simulink model "AlphaBotOdometrie"  (R2026b)
settings: Solver=FixedStepDiscrete  StopTime=inf  FixedStep=PAR_Sys_AbtastBasis_f64  EnableMultiTasking=on
StopFcn:
  | SpeichereOdometrieMessung;
model workspace (MAT data in the model file):
  PAR_AktMot_PWM0_u8 = 80
  PAR_AktMot_RichtL_u8 = 0
  PAR_AktMot_RichtR_u8 = 1
  PAR_AktMot_Start_f32 = Simulink.Parameter
  PAR_AktMot_Start_f32.Value = 0
  PAR_AktMot_Start_f32.Complexity = 'real'
  PAR_AktMot_Start_f32.Dimensions = [1 1]
  PAR_AktMot_Start_f32.DataType = 'single'
  PAR_RegGer_SSoll_f32 = 8
  PAR_SenOdo_IncU_f32 = 40
  PAR_SenOdo_RadR_f32 = 0.0320000015199
  PAR_SenOdo_TTimeout_f32 = 0.20000000298
  PAR_Sys_AbtastBasis_f64 = 0.01
  PAR_Sys_Abtast_f64 = 0.01
libraries: arduinolib x8
settings Model: SILPILModeSetting=veronly  SimulationMode=external
settings SolverCC: AutoInsertRateTranBlk=on
settings DataIOCC: ReturnWorkspaceOutputs=off
settings OptimizationCC: DifferentSizesBufferReuse=on  EfficientTunableParamExpr=on  EnhancedBackFolding=on  MaxStackSize=64  OptimizationCustomize=off  OptimizeBlockOrder=speed  PassReuseOutputArgsAs=Individual arguments  RemoveInternalMemoryZeroInit=on  RemoveRootLevelIOMemoryZeroInit=on
settings DebuggingCC: ParameterTunabilityLossMsg=error
settings HardwareCC: ProdHWDeviceType=ARM Compatible->ARM Cortex  ProdLargestAtomicFloat=Double  ProdLargestAtomicInteger=Long
settings SFSimCC: MATLABDynamicMemAlloc=off
settings RTWCC: BuildConfiguration=Faster Runs  Description=Embedded Coder  HardwareBoard=Arduino Uno R4 WiFi  SystemTargetFile=ert.tlc  TLCOptions=-aInlineSetEventsForThisBaseRateFcn=TLC_FALSE -aSuppressMultiTaskScheduler=TLC_FALSE -aRateBasedStepFcn=1  TemplateMakefile=ert_default_tmf  Toolchain=Arduino ARM M4
settings CodeAppCC: ForceParamTrailComments=on  IgnoreCustomStorageClasses=off  InsertBlockDesc=on  OperatorAnnotations=on  SFDataObjDesc=on  SimulinkDataObjDesc=on
settings ERTTargetCC: CombineSignalStateStructs=on  ExtModeAutomaticAllocSize=off  ExtModeIntrfLevel=Level2 - Open  ExtModeMexFile=ext_xcp  ExtModeStaticAlloc=on  SupportContinuousTime=on  SupportVariableSizeSignals=on

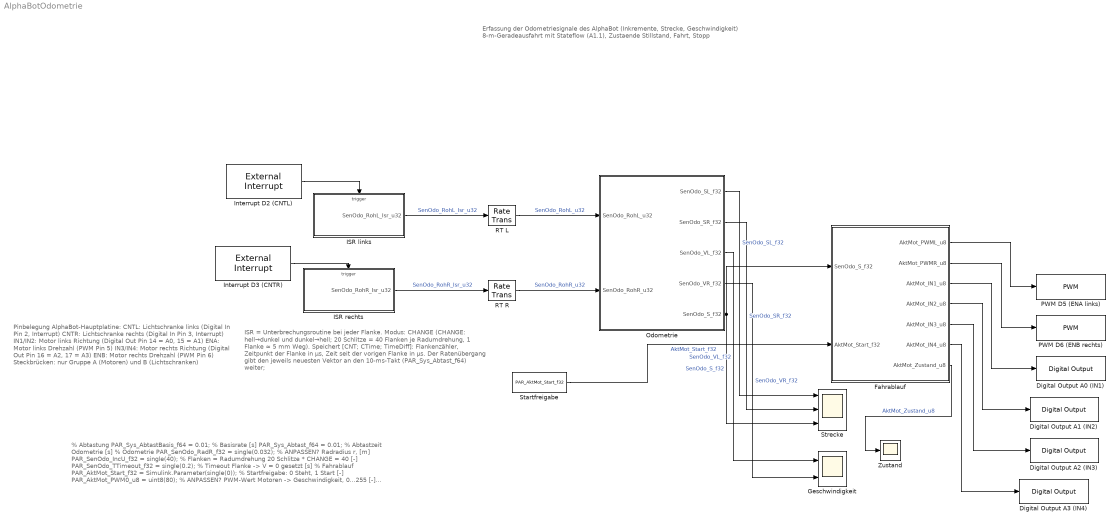
== system AlphaBotOdometrie ==
  note: % Abtastung
      | PAR_Sys_AbtastBasis_f64 = 0.01; % Basisrate [s]
      | PAR_Sys_Abtast_f64 = 0.01; % Abtastzeit Odometrie [s]
      |
      | % Odometrie
      | PAR_SenOdo_RadR_f32 = single(0.032); % ANPASSEN? Radradius r, [m]
      | PAR_SenOdo_IncU_f32 = single(40); % Flanken = Radumdrehung 20 Schlitze * CHANGE = 40 [-]
      | PAR_SenOdo_TTimeout_f32 = single(0.2); % Timeout Flanke -> V = 0 gesetzt [s]
      |
      | % Fahrablauf
      | PAR_AktMot_Start_f32 = Simulink.Parameter(single(0)); % Startfreigabe: 0 Steht, 1 Start [-]
      | PAR_AktMot_PWM0_u8 = uint8(80); % ANPASSEN? PWM-Wert Motoren -> Geschwindigkeit, 0...255 [-]
      | PAR_RegGer_SSoll_f32 = single(8); % Sollstrecke, Fahrt -> Stopp bei S >= SSoll [m]
      | PAR_AktMot_RichtL_u8 = uint8(0); % IN1 (A0) Vorwaertsfahrt links -> IN1 [1]; IN2[0]; IN2 = 1 - IN1 [-]
      | PAR_AktMot_RichtR_u8 = uint8(1); % IN3 (A2) Vorwaertsfahrt rechts; IN4 = 1 - IN3 [-]
      |
      | % Auswertung (analysiereOdometrie.m)
      | S_IST_GEMESSEN = NaN; % ANPASSEN! Referenzwert TOPCON [m]
      | ZEIT_RAND = 2; % ANPASSEN! Stillstand vor/nach Fahrt wegen Zeitachse-Plots[s]
      | TIMEDIFF_MAX = 0.2; % Timeout Flankenabstaende nicht plotten [s]
  note: Erfassung der Odometriesignale des AlphaBot (Inkremente, Strecke, Geschwindigkeit) 8-m-Geradeausfahrt mit Stateflow (A1.1), Zustaende Stillstand, Fahrt, Stopp
  note: Pinbelegung AlphaBot-Hauptplatine:
      | CNTL: Lichtschranke links (Digital In Pin 2, Interrupt)
      | CNTR: Lichtschranke rechts (Digital In Pin 3, Interrupt)
      | IN1/IN2: Motor links Richtung (Digital Out Pin 14 = A0, 15 = A1)
      | ENA: Motor links Drehzahl (PWM Pin 5)
      | IN3/IN4: Motor rechts Richtung (Digital Out Pin 16 = A2, 17 = A3)
      | ENB: Motor rechts Drehzahl (PWM Pin 6)
      | Steckbrücken: nur Gruppe A (Motoren) und B (Lichtschranken)
  note: ISR = Unterbrechungsroutine bei jeder Flanke. Modus: CHANGE
      | (CHANGE: hell→dunkel und dunkel→hell; 20 Schlitze = 40 Flanken je Radumdrehung,
      | 1 Flanke ≈ 5 mm Weg).
      | Speichert [CNT; CTime; TimeDiff]: Flankenzähler, Zeitpunkt der Flanke in µs,
      | Zeit seit der vorigen Flanke in µs.
      | Der Ratenübergang gibt den jeweils neuesten Vektor an den 10-ms-Takt
      | (PAR_Sys_Abtast_f64) weiter;
  Digital Output A0 (IN1) : arduinolib/Digital Output  pinNumber=14  Direction=output  blockPlatform=arduino
  Digital Output A1 (IN2) : arduinolib/Digital Output  pinNumber=15  Direction=output  blockPlatform=arduino
  Digital Output A2 (IN3) : arduinolib/Digital Output  pinNumber=16  Direction=output  blockPlatform=arduino
  Digital Output A3 (IN4) : arduinolib/Digital Output  pinNumber=17  Direction=output  blockPlatform=arduino
  Fahrablauf : Stateflow chart  TreatAsAtomicUnit=on
  Geschwindigkeit : Scope  NumInputPorts=2
      settings: ActiveDisplayYMinimum=-6.2115227592585126E-6  ActiveDisplayYMaximum=5.5903704833326628E-5
  ISR links : Subsystem  TreatAsAtomicUnit=on
  ISR rechts : Subsystem  TreatAsAtomicUnit=on
  Interrupt D2 (CNTL) : arduinolib/External Interrupt  Pin=2  PullUp=off  Mode=CHANGE  InterruptSimulationInput=off
  Interrupt D3 (CNTR) : arduinolib/External Interrupt  Pin=3  PullUp=off  Mode=CHANGE  InterruptSimulationInput=off
  Odometrie : MATLAB Function  TreatAsAtomicUnit=on
  PWM D5 (ENA links) : arduinolib/PWM  pinNumber=5  frequencyType=Default  desiredFrequency=490.2  achievableFrequency=490.2
  PWM D6 (ENB rechts) : arduinolib/PWM  pinNumber=6  frequencyType=Default  desiredFrequency=490.2  achievableFrequency=490.2
  RT L : RateTransition  Deterministic=off  OutPortSampleTime=PAR_Sys_Abtast_f64
  RT R : RateTransition  Deterministic=off  OutPortSampleTime=PAR_Sys_Abtast_f64
  Startfreigabe : Constant  Value=PAR_AktMot_Start_f32  OutDataTypeStr=single  SampleTime=PAR_Sys_Abtast_f64
  Strecke : Scope  NumInputPorts=3
      settings: ActiveDisplayYMinimum=-0.32305176316460693  ActiveDisplayYMaximum=3.1832115141732369
  Zustand : Scope
  wires:
  Interrupt D2 (CNTL)/1 -> ISR links/Trigger
  ISR links/1(SenOdo_RohL_Isr_u32) -> RT L/1  "SenOdo_RohL_Isr_u32"
  Interrupt D3 (CNTR)/1 -> ISR rechts/Trigger
  ISR rechts/1(SenOdo_RohR_Isr_u32) -> RT R/1  "SenOdo_RohR_Isr_u32"
  RT L/1 -> Odometrie/1(SenOdo_RohL_u32)  "SenOdo_RohL_u32"
  RT R/1 -> Odometrie/2(SenOdo_RohR_u32)  "SenOdo_RohR_u32"
  Odometrie/5(SenOdo_S_f32) -> Fahrablauf/1(SenOdo_S_f32), Strecke/3  "SenOdo_S_f32"
  Fahrablauf/1(AktMot_PWML_u8) -> PWM D5 (ENA links)/1
  Fahrablauf/2(AktMot_PWMR_u8) -> PWM D6 (ENB rechts)/1
  Fahrablauf/3(AktMot_IN1_u8) -> Digital Output A0 (IN1)/1
  Fahrablauf/4(AktMot_IN2_u8) -> Digital Output A1 (IN2)/1
  Fahrablauf/5(AktMot_IN3_u8) -> Digital Output A2 (IN3)/1
  Fahrablauf/6(AktMot_IN4_u8) -> Digital Output A3 (IN4)/1
  Odometrie/1(SenOdo_SL_f32) -> Strecke/1  "SenOdo_SL_f32"
  Odometrie/2(SenOdo_SR_f32) -> Strecke/2  "SenOdo_SR_f32"
  Odometrie/3(SenOdo_VL_f32) -> Geschwindigkeit/1  "SenOdo_VL_f32"
  Odometrie/4(SenOdo_VR_f32) -> Geschwindigkeit/2  "SenOdo_VR_f32"
  Fahrablauf/7(AktMot_Zustand_u8) -> Zustand/1  "AktMot_Zustand_u8"
  Startfreigabe/1 -> Fahrablauf/2(AktMot_Start_f32)  "AktMot_Start_f32"

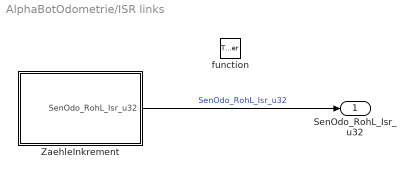
== system AlphaBotOdometrie/ISR links ==
  function : TriggerPort  TriggerType=function-call  VariantControl=(inherit)
  ZaehleInkrement : MATLAB Function  TreatAsAtomicUnit=on
  SenOdo_RohL_Isr_u32 : Outport
  wires:
  ZaehleInkrement/1(SenOdo_RohL_Isr_u32) -> SenOdo_RohL_Isr_u32/1  "SenOdo_RohL_Isr_u32"

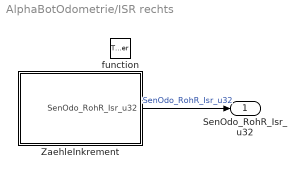
== system AlphaBotOdometrie/ISR rechts ==
  function : TriggerPort  TriggerType=function-call  VariantControl=(inherit)
  ZaehleInkrement : MATLAB Function  TreatAsAtomicUnit=on
  SenOdo_RohR_Isr_u32 : Outport
  wires:
  ZaehleInkrement/1(SenOdo_RohR_Isr_u32) -> SenOdo_RohR_Isr_u32/1  "SenOdo_RohR_Isr_u32"

== matlab function AlphaBotOdometrie/ISR rechts/ZaehleInkrement ==
  data: SenOdo_RohR_Isr_u32 output
function SenOdo_RohR_Isr_u32 = ZaehleInkrement()
% ZaehleInkrement: ISR je Flanke der Lichtschranke (Modus CHANGE)
% Ausgabe:  SenOdo_RohR_Isr_u32 [3x1]: [Flanken seit Programmstart [-]; Zeitstempel micros() [us]; Abstand zur vorigen Flanke [us]]
persistent nZaehler nZeitAlt   % Flankenzaehler [-], Zeitstempel der vorigen Flanke [us]

if isempty(nZaehler)
    nZaehler = uint32(0);
    nZeitAlt = uint32(0);
end
nZeit = uint32(0);   % Zeitstempel dieser Flanke [us]; in der Simulation 0
if coder.target('Rtw')
    coder.cinclude('Arduino.h');
    nZeit = coder.ceval('micros');
end
nZaehler = nZaehler + 1;
SenOdo_RohR_Isr_u32 = [nZaehler; nZeit; nZeit - nZeitAlt];
nZeitAlt = nZeit;
end

== matlab function AlphaBotOdometrie/ISR links/ZaehleInkrement ==
  data: SenOdo_RohL_Isr_u32 output
function SenOdo_RohL_Isr_u32 = ZaehleInkrement()
% ZaehleInkrement: ISR je Flanke der Lichtschranke (Modus CHANGE)
% Ausgabe:  SenOdo_RohL_Isr_u32 [3x1]: [Flanken seit Programmstart [-]; Zeitstempel micros() [us]; Abstand zur vorigen Flanke [us]]
persistent nZaehler nZeitAlt   % Flankenzaehler [-], Zeitstempel der vorigen Flanke [us]

if isempty(nZaehler)
    nZaehler = uint32(0);
    nZeitAlt = uint32(0);
end
nZeit = uint32(0);   % Zeitstempel dieser Flanke [us]; in der Simulation 0
if coder.target('Rtw')
    coder.cinclude('Arduino.h');
    nZeit = coder.ceval('micros');
end
nZaehler = nZaehler + 1;
SenOdo_RohL_Isr_u32 = [nZaehler; nZeit; nZeit - nZeitAlt];
nZeitAlt = nZeit;
end

== matlab function AlphaBotOdometrie/Odometrie ==
  settings: updateMethod=DISCRETE  sampleTime=PAR_Sys_Abtast_f64
  data: SenOdo_RohL_u32 input; SenOdo_SL_f32 output; SenOdo_RohR_u32 input; SenOdo_SR_f32 output; SenOdo_VL_f32 output; SenOdo_VR_f32 output; SenOdo_S_f32 output; PAR_SenOdo_RadR_f32 parameter; PAR_SenOdo_IncU_f32 parameter; PAR_SenOdo_TTimeout_f32 parameter; PAR_Sys_Abtast_f64 parameter
function [SenOdo_SL_f32,SenOdo_SR_f32,SenOdo_VL_f32,SenOdo_VR_f32,SenOdo_S_f32] = BerechneOdometrie(SenOdo_RohL_u32,SenOdo_RohR_u32,PAR_SenOdo_RadR_f32, PAR_SenOdo_IncU_f32, PAR_SenOdo_TTimeout_f32, PAR_Sys_Abtast_f64)
% BerechneOdometrie: Strecke und Geschwindigkeit je Rad aus Flankenzaehler und Flankenabstand
% Radachse Lochscheibe mit 20 Schlitzen. Jeder Wechsel hell/dunkel ist eine "Flanke"; pro Radumdrehung 
% 40 Flanken. ISR zaehlt Flanken und Zeit -> Block laeuft alle PAR_Sys_Abtast_f64 = 0,01 s   
%     Strecke        = Anzahl Flanken * Weg je Flanke
%     Geschwindigkeit = Weg je Flanke / Zeit zwischen den letzten zwei Flanken
%
% Eingabe:  SenOdo_RohL_u32,        Signal PhotoSensor L
%           SenOdo_RohR_u32,        Signal PhotoSensor L
%           PAR_SenOdo_RadR_f32     Radradius r
%           PAR_SenOdo_IncU_f32     Flanken je Radumdrehung
%           PAR_SenOdo_TTimeout_f32 Zeit ohne Flanke, V = 0 gesetzt wird [s] 
%           PAR_Sys_Abtast_f64      Abtastzeit dieses Blocks [s] (0,01 s)
% Ausgabe:  SenOdo_SL_f32, SenOdo_SR_f32 [1x1]: Radstrecke links, rechts [m]
%           SenOdo_VL_f32, SenOdo_VR_f32 [1x1]: Radgeschwindigkeit links, rechts [m/s]
%           SenOdo_S_f32                 [1x1]: mittlere Strecke des Roboters [m]

persistent anZaehlerAlt afZeitOhne   % Zaehlerstand im vorigen Schritt [-], Zeit seit der letzten Flanke [s]

if isempty(anZaehlerAlt)
    anZaehlerAlt = zeros(2,1,'uint32');
    afZeitOhne = zeros(2,1,'single');
end

% Weg je Flanke: 2*pi*r/40 ~5mm je Flanke
fWegInkrement = 2 * single(pi) * PAR_SenOdo_RadR_f32 / PAR_SenOdo_IncU_f32;   % Weg je Flanke [m]

anZaehler = [SenOdo_RohL_u32(1); SenOdo_RohR_u32(1)];   % Flankenzaehler links, rechts [-]

% Mikrosekunden in Sekunden umrechnen(Faktor 1e-6).
afAbstand = single([SenOdo_RohL_u32(end); SenOdo_RohR_u32(end)]) * single(1e-6);   % Flankenabstand [s]
afGeschw = zeros(2,1,'single');   % Radgeschwindigkeit links, rechts [m/s]

% Geschwindigkeit je Rad (k = 1 links, k = 2 rechts):
for k = 1:2
    if anZaehler(k) ~= anZaehlerAlt(k)

        % Zaehler hat sich seit dem letzten Aufruf geaendert: Rad dreht, Uhr zuruecksetzen
        afZeitOhne(k) = 0;

    elseif afZeitOhne(k) < PAR_SenOdo_TTimeout_f32

        % keine neue Flanke: Wartezeit um eine Abtastzeit (0,01 s) erhoehen,
        afZeitOhne(k) = afZeitOhne(k) + single(PAR_Sys_Abtast_f64);

    end

    if afZeitOhne(k) < PAR_SenOdo_TTimeout_f32 && afAbstand(k) > 0
        afGeschw(k) = fWegInkrement / afAbstand(k);
    end
end

anZaehlerAlt = anZaehler;

% Strecke je Rad = Anzahl Flanken * Weg je Flanke.
afStrecke = single(anZaehler) * fWegInkrement;   % Radstrecke links, rechts [m]

% Ergebnisse Ausgaenge verteilen
SenOdo_SL_f32 = afStrecke(1);
SenOdo_SR_f32 = afStrecke(2);
SenOdo_VL_f32 = afGeschw(1);
SenOdo_VR_f32 = afGeschw(2);
% Mittlere Strecke des Roboters s = (sL + sR) / 2; der Stateflow-Chart stoppt bei s >= PAR_RegGer_SSoll_f32 (8 m)
SenOdo_S_f32 = (afStrecke(1) + afStrecke(2)) / 2;
end

% Grenzen (fuer die Auswertung wichtig):
% - Aufloesung: Strecke nur in Schritten von etwa 5 mm.
% - V aus einer einzigen Flanke ist unruhig: Schlitz und Steg der Scheibe sind
%   ungleich breit, TimeDiff wechselt zwischen kurz und lang (Vorgabedaten: V etwa 3,9-mal
%   zu hoch). Zuverlaessiger ist die mittlere Geschwindigkeit aus der Strecke.
% - Keine Drehrichtung: rueckwaerts wird ebenfalls aufwaerts gezaehlt.
% - Falscher Radradius verfaelscht S und V im selben Verhaeltnis (z. B. r 1 mm zu klein:
%   etwa 3 % zu wenig Strecke).

== stateflow chart AlphaBotOdometrie/Fahrablauf ==
  settings: updateMethod=DISCRETE  sampleTime=PAR_Sys_Abtast_f64  executeAtInitialization=1
  note: Stateflow-Chart Fahrablauf (Ablaufsteuerung, Abtastzeit PAR_Sys_Abtast_f64 = 0,01 s)
      |
      | Zustände (AktMot_Zustand_u8):
      | 0 Stillstand: alle PWM- und Richtungsausgänge 0 -> Motoren aus, Warten auf Start.
      | 1 Fahrt2m:    PWM L/R = PAR_AktMot_PWM0_u8 (80 von 255), Richtungspins vorwärts.
      | 2 Stopp:      alle Ausgänge 0. Endzustand, kein Rückweg; Neustart nur durch Neustart des Programms.
      |
      | Übergänge:
      | Start:  PAR_AktMot_Start_f32 per Monitor & Tune von 0 auf 1 (Constant "Startfreigabe" -> AktMot_Start_f32).
      | Ziel:   s = (S_L + S_R)/2 >= 2 m;  S_L,R = CNT_L,R * 2*pi*r/40  (r = 0,032 m -> ca. 5 mm je Flanke, 2 m ~ 398 Flanken).
      |
      | Richtung (L298P: Motor dreht nur bei IN1 ungleich IN2):
      | IN1 = PAR_AktMot_RichtL_u8 (0), IN2 = 1 - IN1 (1)   -> Motor links vorwärts
      | IN3 = PAR_AktMot_RichtR_u8 (1), IN4 = 1 - IN3 (0)   -> Motor rechts vorwärts (spiegelbildlich eingebaut)
      |
      | Ausgänge: AktMot_PWML_u8/PWMR_u8 -> PWM D5/D6; AktMot_IN1..IN4_u8 -> Digital Output A0..A3 (Pins 14..17);
  state Fahrt
    entry:
    AktMot_PWML_u8 = PAR_AktMot_PWM0_u8;
    AktMot_PWMR_u8 = PAR_AktMot_PWM0_u8;
    AktMot_IN1_u8 = PAR_AktMot_RichtL_u8;
    AktMot_IN2_u8 = uint8(1) - PAR_AktMot_RichtL_u8;
    AktMot_IN3_u8 = PAR_AktMot_RichtR_u8;
    AktMot_IN4_u8 = uint8(1) - PAR_AktMot_RichtR_u8;
    AktMot_Zustand_u8 = uint8(1);
  state Stopp
    entry:
    AktMot_PWML_u8 = uint8(0);
    AktMot_PWMR_u8 = uint8(0);
    AktMot_IN1_u8 = uint8(0);
    AktMot_IN2_u8 = uint8(0);
    AktMot_IN3_u8 = uint8(0);
    AktMot_IN4_u8 = uint8(0);
    AktMot_Zustand_u8 = uint8(2);
  state Stillstand
    entry:
    AktMot_PWML_u8 = uint8(0);
    AktMot_PWMR_u8 = uint8(0);
    AktMot_IN1_u8 = uint8(0);
    AktMot_IN2_u8 = uint8(0);
    AktMot_IN3_u8 = uint8(0);
    AktMot_IN4_u8 = uint8(0);
    AktMot_Zustand_u8 = uint8(0);
  (default) -> Stillstand
  Fahrt -> Stopp : [SenOdo_S_f32 >= PAR_RegGer_SSoll_f32]
  Stillstand -> Fahrt : [AktMot_Start_f32 >= 1]
  data: SenOdo_S_f32 input single; AktMot_Start_f32 input single; AktMot_PWML_u8 output uint8; AktMot_PWMR_u8 output uint8; AktMot_IN1_u8 output uint8; AktMot_IN2_u8 output uint8; AktMot_IN3_u8 output uint8; AktMot_IN4_u8 output uint8; PAR_AktMot_PWM0_u8 parameter uint8; PAR_RegGer_SSoll_f32 parameter single; PAR_AktMot_RichtL_u8 parameter uint8; PAR_AktMot_RichtR_u8 parameter uint8; AktMot_Zustand_u8 output uint8
